simulink model "ParkTransforms"  (R2026b)
settings: Solver=VariableStepAuto
settings Model: Creator=24322  LastModifiedBy=24322

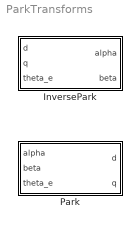
== system ParkTransforms ==
  InversePark : Subsystem
  Park : Subsystem

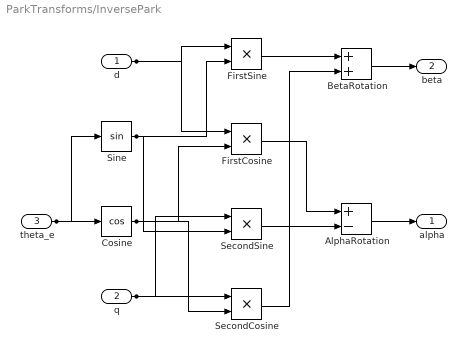
== system ParkTransforms/InversePark ==
  d : Inport  OutDataTypeStr=double
  q : Inport  Port=2  OutDataTypeStr=double
  theta_e : Inport  Port=3  OutDataTypeStr=double
  AlphaRotation : Sum  Inputs=+-
  BetaRotation : Sum
  Cosine : Trigonometry  Operator=cos
  FirstCosine : Product  Inputs=**
  FirstSine : Product  Inputs=**
  SecondCosine : Product  Inputs=**
  SecondSine : Product  Inputs=**
  Sine : Trigonometry
  alpha : Outport
  beta : Outport  Port=2
  wires:
  BetaRotation/1 -> beta/1
  AlphaRotation/1 -> alpha/1
  SecondCosine/1 -> BetaRotation/2
  FirstSine/1 -> BetaRotation/1
  SecondSine/1 -> AlphaRotation/2
  FirstCosine/1 -> AlphaRotation/1
  q/1 -> SecondCosine/1, SecondSine/1
  Sine/1 -> FirstSine/2, SecondSine/2
  Cosine/1 -> FirstCosine/2, SecondCosine/2
  d/1 -> FirstCosine/1, FirstSine/1
  theta_e/1 -> Cosine/1, Sine/1

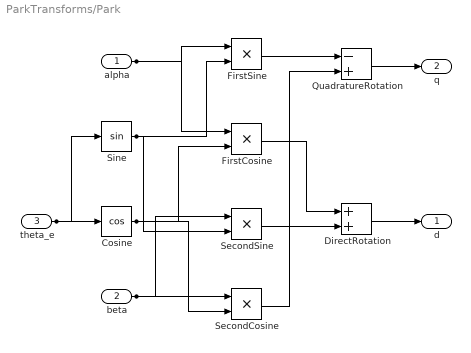
== system ParkTransforms/Park ==
  alpha : Inport  OutDataTypeStr=double
  beta : Inport  Port=2  OutDataTypeStr=double
  theta_e : Inport  Port=3  OutDataTypeStr=double
  Cosine : Trigonometry  Operator=cos
  DirectRotation : Sum
  FirstCosine : Product  Inputs=**
  FirstSine : Product  Inputs=**
  QuadratureRotation : Sum  Inputs=-+
  SecondCosine : Product  Inputs=**
  SecondSine : Product  Inputs=**
  Sine : Trigonometry
  d : Outport
  q : Outport  Port=2
  wires:
  QuadratureRotation/1 -> q/1
  DirectRotation/1 -> d/1
  SecondCosine/1 -> QuadratureRotation/2
  FirstSine/1 -> QuadratureRotation/1
  SecondSine/1 -> DirectRotation/2
  FirstCosine/1 -> DirectRotation/1
  beta/1 -> SecondCosine/1, SecondSine/1
  Sine/1 -> FirstSine/2, SecondSine/2
  Cosine/1 -> FirstCosine/2, SecondCosine/2
  alpha/1 -> FirstCosine/1, FirstSine/1
  theta_e/1 -> Cosine/1, Sine/1
